simulink model "emso1"  (Simulink 7.1)
settings: Solver=ode45  StartTime=0.0  StopTime=5  RelTol=1e-3
settings Model: Creator=lades  LastModifiedBy=Administrador
settings DataIOCC: ExternalInput=Az
settings DebuggingCC: SaveWithDisabledLinksMsg=none  SaveWithParameterizedLinksMsg=none  CheckSSInitialOutputMsg=off  SolverPrmCheckMsg=none  MultiTaskCondExecSysMsg=none  Int32ToFloatConvMsg=none  ModelReferenceDataLoggingMessage=none

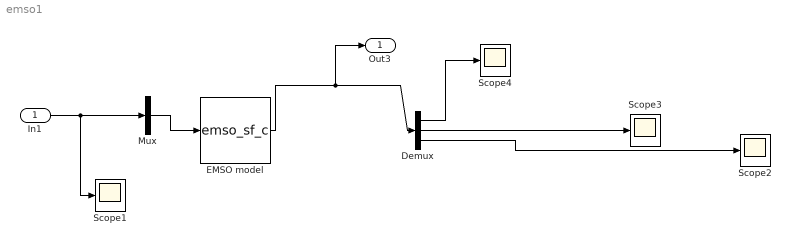
== system emso1 ==
  In1 : Inport
  Demux : Demux  Outputs=3
  EMSO model : S-Function  FunctionName=emso_sf_c  Parameters='Problem_2F.ems',4,3  EnableBusSupport=off
  Mux : Mux  Inputs=1
  Scope{1..4} (4 alike) : Scope
      Scope1 settings: TimeRange=2  YMin=4.008258966500001  YMax=4.008258969500001
      Scope2 settings: TimeRange=5  YMin=0  YMax=45
      Scope3 settings: TimeRange=5  YMin=0  YMax=45  SaveName=ScopeData2
      Scope4 settings: TimeRange=5  YMin=0  YMax=45  SaveName=ScopeData3
  Out3 : Outport
  wires:
  EMSO model/1 -> Demux/1, Out3/1
  Mux/1 -> EMSO model/1
  In1/1 -> Mux/1, Scope1/1
  Demux/3 -> Scope2/1
  Demux/2 -> Scope3/1
  Demux/1 -> Scope4/1
